simulink model "ball_balancing_omni3_stm32_lqi_rev1"  (R2024b)
settings: Solver=FixedStepDiscrete  StartTime=0.0  StopTime=5  FixedStep=ballbotParams.controller.sampleTime  RelTol=1e-3
PreLoadFcn:
  | if ~exist('ballbotParams','var'), ballbotParams = ballbotRev1Parameters; end
InitFcn:
  | if ~exist('ballbotParams','var') || ~isfield(ballbotParams,'parameterSource') || ballbotParams.parameterSource ~= "ballbotRev1Parameters" || ~isfield(ballbotParams,'controller') || ~isfield(ballbotParams,'estimator'), ballbotParams = ballbotRev1Parameters; end
  | clear functions;
undefined symbols (not defined in the file or in its folder): ballbotEstimatorInitialState, ballbotEstimatorUpdate, ballbotLqiControllerUpdate, ballbotParams, ballbotTorqueDutyStep, ballbotWheelRateFromDisplacement
settings Model: Creator=cafdr  LastModifiedBy=cafdr
settings ModelReferenceCC: UpdateModelReferenceTargets=IfOutOfDate
settings ConfigComp: CovBoundaryAbsTol=1.0e-5

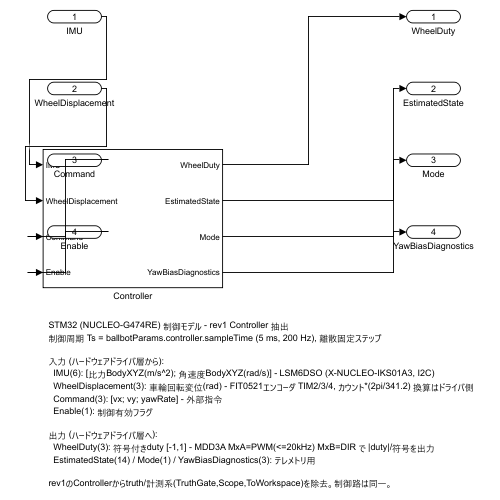
[thumbnail: Simulink's stored preview of the top-level diagram]
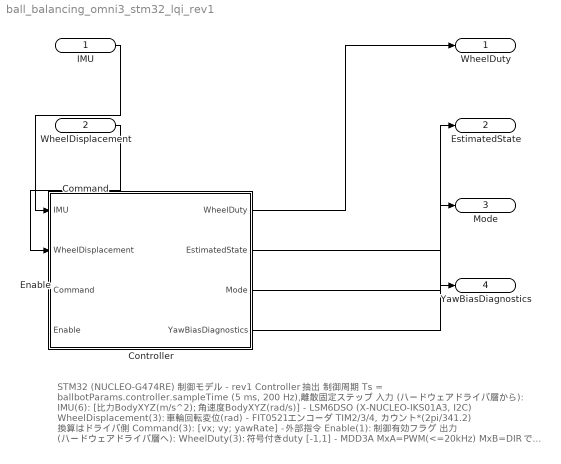
== system ball_balancing_omni3_stm32_lqi_rev1 ==
  note: STM32 (NUCLEO-G474RE) 制御モデル - rev1 Controller 抽出
      | 制御周期 Ts = ballbotParams.controller.sampleTime (5 ms, 200 Hz), 離散固定ステップ
      |
      | 入力 (ハードウェアドライバ層から):
      |   IMU(6): [比力BodyXYZ(m/s^2); 角速度BodyXYZ(rad/s)] - LSM6DSO (X-NUCLEO-IKS01A3, I2C)
      |   WheelDisplacement(3): 車輪回転変位(rad) - FIT0521エンコーダ TIM2/3/4, カウント*(2pi/341.2) 換算はドライバ側
      |   Command(3): [vx; vy; yawRate] - 外部指令
      |   Enable(1): 制御有効フラグ
      |
      | 出力 (ハードウェアドライバ層へ):
      |   WheelDuty(3): 符号付きduty [-1,1] - MDD3A MxA=PWM(<=20kHz) MxB=DIR で |duty|/符号を出力
      |   EstimatedState(14) / Mode(1) / YawBiasDiagnostics(3): テレメトリ用
      |
      | rev1のControllerからtruth/計測系(TruthGate,Scope,ToWorkspace)を除去。制御路は同一。
  IMU : Inport
  WheelDisplacement : Inport  Port=2
  Command : Inport  Port=3
  Enable : Inport  Port=4
  Controller : Subsystem
  WheelDuty : Outport
  EstimatedState : Outport  Port=2
  Mode : Outport  Port=3
  YawBiasDiagnostics : Outport  Port=4
  wires:
  Controller/1(WheelDuty) -> WheelDuty/1
  Controller/2(EstimatedState) -> EstimatedState/1
  Controller/3(Mode) -> Mode/1
  Controller/4(YawBiasDiagnostics) -> YawBiasDiagnostics/1
  IMU/1 -> Controller/1(IMU)
  WheelDisplacement/1 -> Controller/2(WheelDisplacement)
  Command/1 -> Controller/3(Command)
  Enable/1 -> Controller/4(Enable)

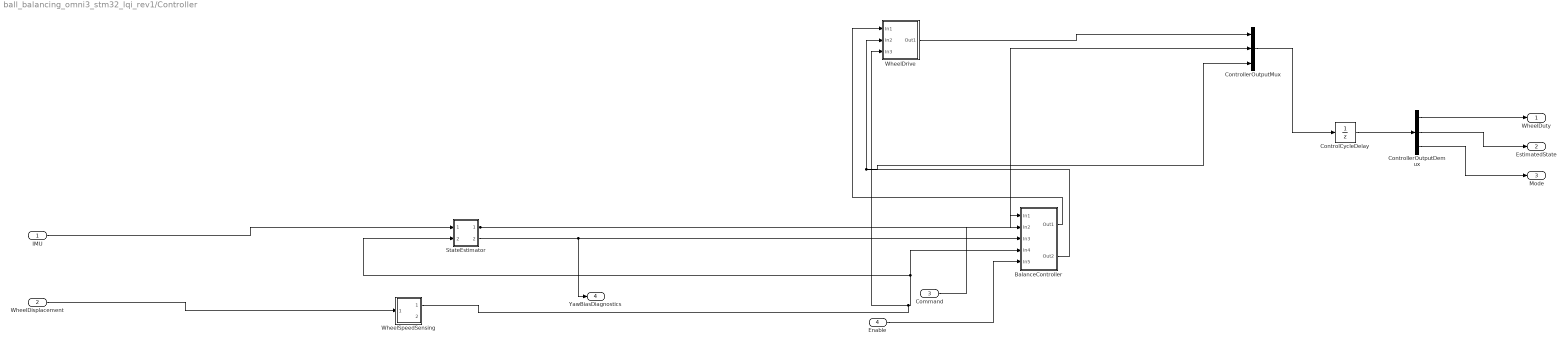
== system ball_balancing_omni3_stm32_lqi_rev1/Controller ==
  IMU : Inport  PortDimensions=6
  WheelDisplacement : Inport  Port=2  PortDimensions=3
  Command : Inport  Port=3
  Enable : Inport  Port=4
  BalanceController : Subsystem
  ControlCycleDelay : UnitDelay  InitialCondition=zeros(18,1)  SampleTime=ballbotParams.controller.sampleTime
  ControllerOutputDemux : Demux  Outputs=[3 14 1]
  ControllerOutputMux : Mux  Inputs=3
  StateEstimator : Subsystem
  WheelDrive : Subsystem
  WheelSpeedSensing : Subsystem
  WheelDuty : Outport
  EstimatedState : Outport  Port=2
  Mode : Outport  Port=3
  YawBiasDiagnostics : Outport  Port=4
  wires:
  WheelDrive/1(Out1) -> ControllerOutputMux/1
  Enable/1 -> BalanceController/5(In5)
  Command/1 -> BalanceController/2(In2)
  BalanceController/2(Out2) -> ControllerOutputMux/3, WheelDrive/2(In2)
  BalanceController/1(Out1) -> WheelDrive/1(In1)
  IMU/1 -> StateEstimator/1(In1)
  StateEstimator/2(Out2) -> BalanceController/3(In3), YawBiasDiagnostics/1
  WheelDisplacement/1 -> WheelSpeedSensing/1(In1)
  WheelSpeedSensing/1(Out1) -> WheelDrive/3(In3), StateEstimator/2(In2), BalanceController/4(In4)
  ControllerOutputMux/1 -> ControlCycleDelay/1
  ControllerOutputDemux/2 -> EstimatedState/1
  ControllerOutputDemux/1 -> WheelDuty/1
  ControllerOutputDemux/3 -> Mode/1
  ControlCycleDelay/1 -> ControllerOutputDemux/1
  StateEstimator/1(Out1) -> BalanceController/1(In1), ControllerOutputMux/2

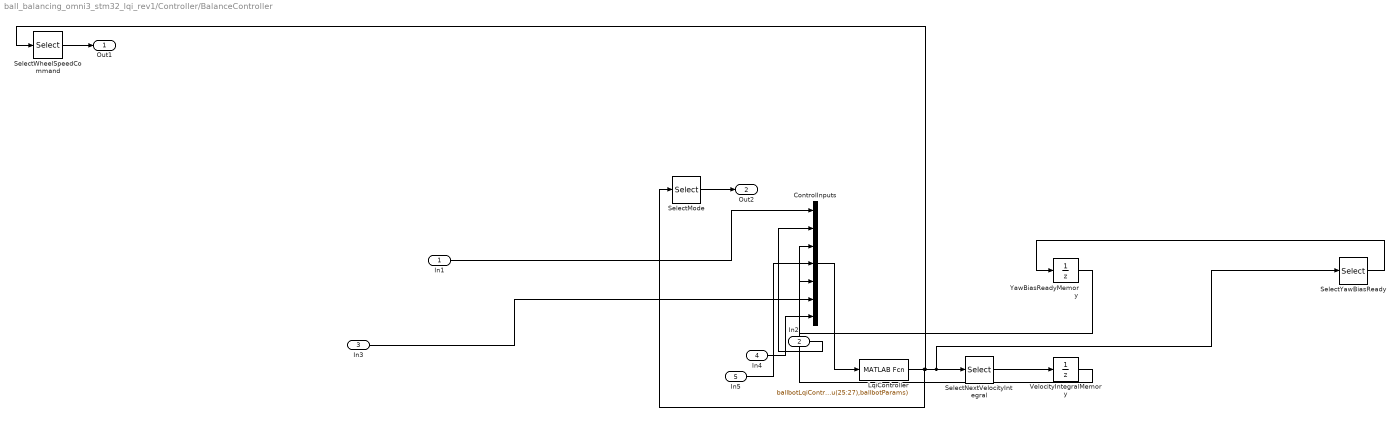
== system ball_balancing_omni3_stm32_lqi_rev1/Controller/BalanceController ==
  In1 : Inport
  In2 : Inport  Port=2
  In3 : Inport  Port=3
  In4 : Inport  Port=4
  In5 : Inport  Port=5
  ControlInputs : Mux  Inputs=7
  LqiController : MATLABFcn  MATLABFcn=ballbotLqiControllerUpdate(u(1:14),u(15:17),u(18:19),u(20),u(21),u(22:24),u(25:27),ballbotParams)  OutputDimensions=7  SampleTime=ballbotParams.controller.sampleTime
  SelectMode : Selector  InputPortWidth=7  IndexOptions=Index vector (dialog)  Indices=6  OutputSizes=1
  SelectNextVelocityIntegral : Selector  InputPortWidth=7  IndexOptions=Index vector (dialog)  Indices=4:5  OutputSizes=1
  SelectWheelSpeedCommand : Selector  InputPortWidth=7  IndexOptions=Index vector (dialog)  Indices=1:3  OutputSizes=1
  SelectYawBiasReady : Selector  InputPortWidth=7  IndexOptions=Index vector (dialog)  Indices=7  OutputSizes=1
  VelocityIntegralMemory : UnitDelay  InitialCondition=zeros(2,1)  SampleTime=ballbotParams.controller.sampleTime
  YawBiasReadyMemory : UnitDelay  SampleTime=ballbotParams.controller.sampleTime
  Out1 : Outport
  Out2 : Outport  Port=2
  wires:
  In2/1 -> ControlInputs/2
  SelectMode/1 -> Out2/1
  In4/1 -> ControlInputs/7
  In5/1 -> ControlInputs/4
  ControlInputs/1 -> LqiController/1
  In3/1 -> ControlInputs/6
  SelectWheelSpeedCommand/1 -> Out1/1
  YawBiasReadyMemory/1 -> ControlInputs/5
  SelectYawBiasReady/1 -> YawBiasReadyMemory/1
  VelocityIntegralMemory/1 -> ControlInputs/3
  In1/1 -> ControlInputs/1
  LqiController/1 -> SelectMode/1, SelectWheelSpeedCommand/1, SelectNextVelocityIntegral/1, SelectYawBiasReady/1
  SelectNextVelocityIntegral/1 -> VelocityIntegralMemory/1

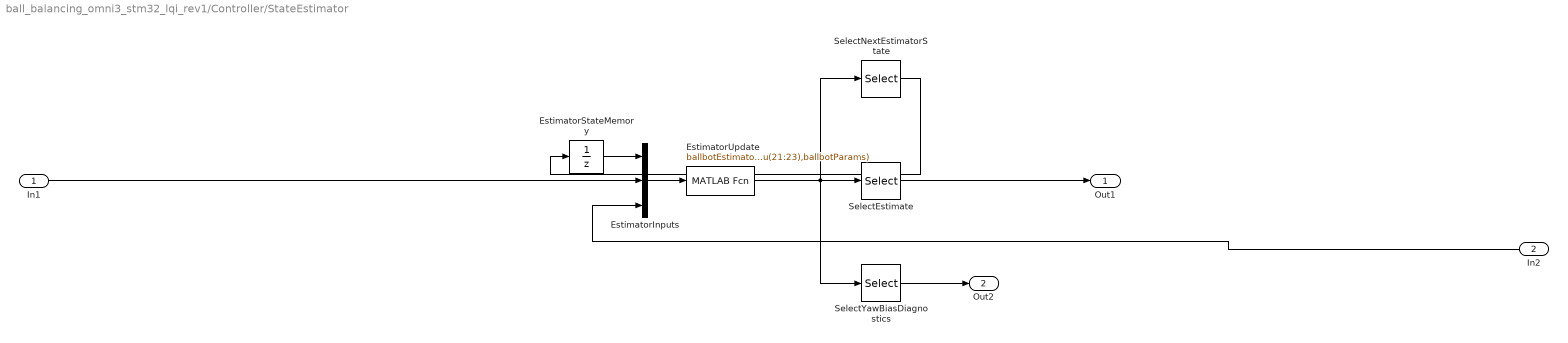
== system ball_balancing_omni3_stm32_lqi_rev1/Controller/StateEstimator ==
  In1 : Inport
  In2 : Inport  Port=2
  EstimatorInputs : Mux  Inputs=3
  EstimatorStateMemory : UnitDelay  InitialCondition=ballbotEstimatorInitialState(ballbotParams)  SampleTime=ballbotParams.controller.sampleTime
  EstimatorUpdate : MATLABFcn  MATLABFcn=ballbotEstimatorUpdate(u(1:14),u(15:20),u(21:23),ballbotParams)  OutputDimensions=31  SampleTime=ballbotParams.controller.sampleTime
  SelectEstimate : Selector  InputPortWidth=31  IndexOptions=Index vector (dialog)  Indices=15:28  OutputSizes=1
  SelectNextEstimatorState : Selector  InputPortWidth=31  IndexOptions=Index vector (dialog)  Indices=1:14  OutputSizes=1
  SelectYawBiasDiagnostics : Selector  InputPortWidth=31  IndexOptions=Index vector (dialog)  Indices=29:31  OutputSizes=1
  Out1 : Outport
  Out2 : Outport  Port=2
  wires:
  In1/1 -> EstimatorInputs/2
  EstimatorInputs/1 -> EstimatorUpdate/1
  SelectEstimate/1 -> Out1/1
  EstimatorStateMemory/1 -> EstimatorInputs/1
  SelectNextEstimatorState/1 -> EstimatorStateMemory/1
  In2/1 -> EstimatorInputs/3
  EstimatorUpdate/1 -> SelectYawBiasDiagnostics/1, SelectNextEstimatorState/1, SelectEstimate/1
  SelectYawBiasDiagnostics/1 -> Out2/1

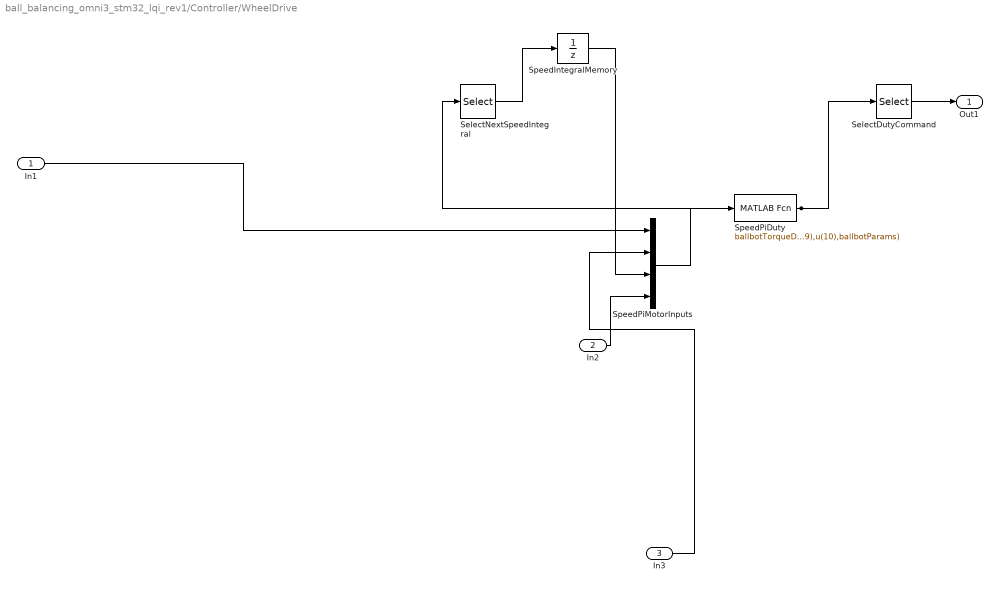
== system ball_balancing_omni3_stm32_lqi_rev1/Controller/WheelDrive ==
  In1 : Inport
  In2 : Inport  Port=2
  In3 : Inport  Port=3
  SelectDutyCommand : Selector  InputPortWidth=6  IndexOptions=Index vector (dialog)  Indices=1:3  OutputSizes=1
  SelectNextSpeedIntegral : Selector  InputPortWidth=6  IndexOptions=Index vector (dialog)  Indices=4:6  OutputSizes=1
  SpeedIntegralMemory : UnitDelay  InitialCondition=zeros(3,1)  SampleTime=ballbotParams.controller.sampleTime
  SpeedPiDuty : MATLABFcn  MATLABFcn=ballbotTorqueDutyStep(u(1:3),u(4:6),u(7:9),u(10),ballbotParams)  OutputDimensions=6  SampleTime=ballbotParams.controller.sampleTime
  SpeedPiMotorInputs : Mux
  Out1 : Outport
  wires:
  In3/1 -> SpeedPiMotorInputs/2
  SpeedIntegralMemory/1 -> SpeedPiMotorInputs/3
  In1/1 -> SpeedPiMotorInputs/1
  In2/1 -> SpeedPiMotorInputs/4
  SelectDutyCommand/1 -> Out1/1
  SpeedPiDuty/1 -> SelectNextSpeedIntegral/1, SelectDutyCommand/1
  SpeedPiMotorInputs/1 -> SpeedPiDuty/1
  SelectNextSpeedIntegral/1 -> SpeedIntegralMemory/1

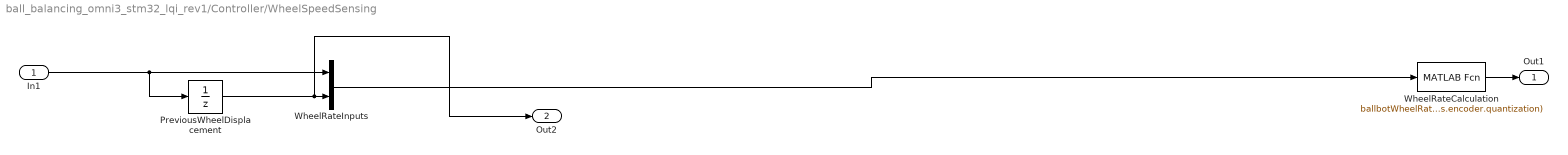
== system ball_balancing_omni3_stm32_lqi_rev1/Controller/WheelSpeedSensing ==
  In1 : Inport
  PreviousWheelDisplacement : UnitDelay  InitialCondition=zeros(3,1)  SampleTime=ballbotParams.controller.sampleTime
  WheelRateCalculation : MATLABFcn  MATLABFcn=ballbotWheelRateFromDisplacement(u(1:3),u(4:6),ballbotParams.estimator.sampleTime,ballbotParams.encoder.quantization)  OutputDimensions=3  SampleTime=ballbotParams.controller.sampleTime
  WheelRateInputs : Mux  Inputs=2
  Out1 : Outport
  Out2 : Outport  Port=2
  wires:
  PreviousWheelDisplacement/1 -> WheelRateInputs/2, Out2/1
  WheelRateInputs/1 -> WheelRateCalculation/1
  WheelRateCalculation/1 -> Out1/1
  In1/1 -> PreviousWheelDisplacement/1, WheelRateInputs/1
